simulink model "DPWMA_17_Level_Rectifier_Digital_PR"  (R2023b)
settings: Solver=VariableStepAuto  StartTime=0.0  StopTime=0.5  RelTol=1e-3
libraries: spsDiodeLib x144, spsSeriesRLCBranchLib x39, spsVoltageMeasurementLib x27, spsIGBTDiodeLib x24, simulink x12, spsACVoltageSourceLib x3, spsCurrentMeasurementLib x2, spsMeanLib x2, spsRMSLib x2, slpidlib x1, spsTHDLib x1, spspowerguiLib x1
(part 1 of 2)
settings Model: SimulationMode=accelerator  Creator=abc68  LastModifiedBy=Qu
settings DebuggingCC: UnconnectedInputMsg=warning  UnconnectedOutputMsg=warning  UnconnectedLineMsg=warning
settings ModelReferenceCC: EnableRefExpFcnMdlSchedulingChecks=on
settings RTWCC: DLArmComputeVersion=19.05

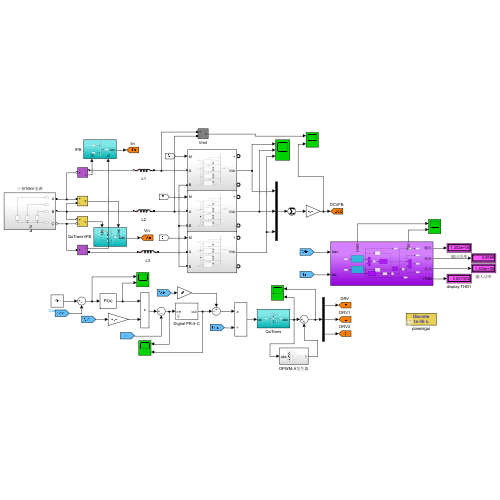
[thumbnail: Simulink's stored preview of the top-level diagram]
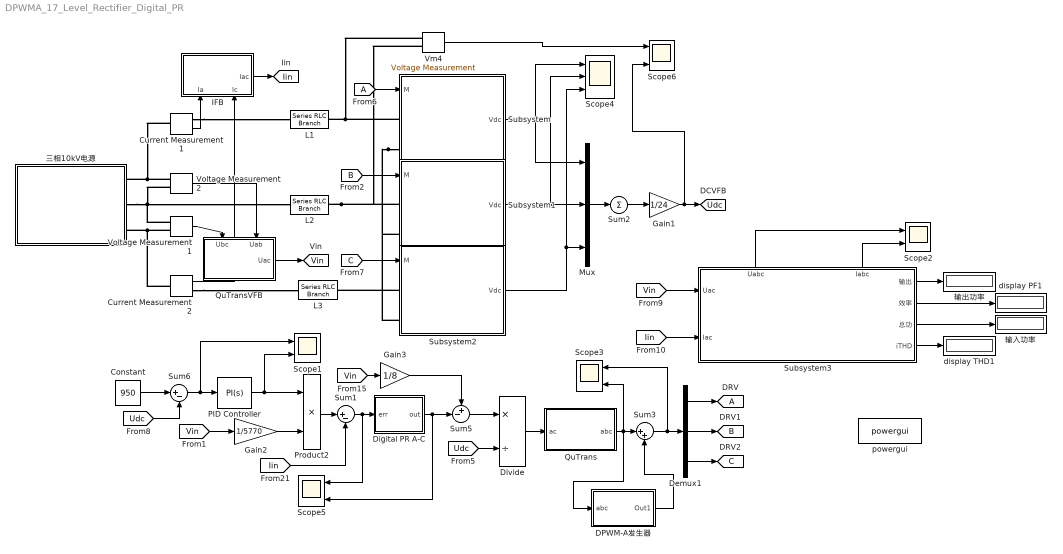
== system DPWMA_17_Level_Rectifier_Digital_PR ==
  Constant : Constant  Value=950
  Current Measurement1 : spsCurrentMeasurementLib/Current Measurement  PhasorSimulation=off  OutputType=Complex  PSBequivalent=0
  Current Measurement2 : spsCurrentMeasurementLib/Current Measurement  PhasorSimulation=off  OutputType=Complex  PSBequivalent=0
  DPWM-A发生器 : Subsystem
  DRV : Goto  TagVisibility=global
  Demux1 : Demux  Outputs=3
  Digital PR A-C : Subsystem  mask{Kp=3, Kr=30, Wc=5, Ts=1/28800, Upper=3000, Lower=-3000}
      mask DialogControl ParameterGroupVar Prompt: 参数
  Divide : Product  Inputs=*/
  From6 : From  TagVisibility=global
  Gain1 : Gain  Gain=1/24
  Gain2 : Gain  Gain=1/5770
  Gain3 : Gain  Gain=1/8
  IFB : Subsystem
      settings: PortSchema="{\"entries\":[{\"content\":{\"sides\":[{\"content\":{\"connectorIds\":[]},\"type\":\"ConnectorPlacement.EquallySpacedRectSide\",\"uuid\":\"58c40194-9a95-4e39-952e-f878bde7484e\"},{\"content\":{\"connectorIds\":[\"In1\",\"In2\"],\"side\":\"RIGHT\"},\"type\":\"ConnectorPlacement.EquallySpacedRectSide\",\"uuid\":\"f51692e8-3ff2-4d72-808d-3667196a4526\"},{\"content\":{\"connectorIds\":[],\"side\":\"TOP\"},\"type\":\"ConnectorPlacement.EquallySpacedRectSide\",\"uuid\":\"0aab136b-5da5-45c4-8998-999ebe8b7f2f\"},{\"content\":{\"connectorIds\":[\"Out1\"],\"side\":\"BOTTOM\"},\"type\":\"ConnectorPlacement.EquallySpacedRectSide\",\"uuid\":\"32f5f4a5-4ebb-496b-828d-b973bd46b44e\"}]},\"type\":\"ConnectorPlacement.EquallySpacedConnector\",\"uuid\":\"3ef81af7-d426-47fb-88e3-e33e58eebb83\"}],\"packageUris\":[\"http://schema.mathworks.com/mf0/Connector/R2020b\"],\"version\":\"1.0\"}"
  L1 : spsSeriesRLCBranchLib/Series RLC Branch  LConnTagsString=__new0  RConnTagsString=__new0  BranchType=L  Resistance=0.05  Inductance=5e-3  SetiL0=off  InitialCurrent=0  Capacitance=inf  Setx0=off  InitialVoltage=0  Measurements=None
  L2 : spsSeriesRLCBranchLib/Series RLC Branch  LConnTagsString=__new0  RConnTagsString=__new0  BranchType=L  Resistance=0.05  Inductance=5e-3  SetiL0=off  InitialCurrent=0  Capacitance=inf  Setx0=off  InitialVoltage=0  Measurements=None
  L3 : spsSeriesRLCBranchLib/Series RLC Branch  LConnTagsString=__new0  RConnTagsString=__new0  BranchType=L  Resistance=0.05  Inductance=5e-3  SetiL0=off  InitialCurrent=0  Capacitance=inf  Setx0=off  InitialVoltage=0  Measurements=None
  Mux : Mux  Inputs=3
  PID Controller : slpidlib/PID Controller  Controller=PI  Form=Parallel  TimeDomain=Continuous-time  UseExternalTs=off  SampleTime=-1  IntegratorMethod=Forward Euler  FilterMethod=Forward Euler  ControllerParametersSource=internal  P=1.5  I=120  UseKiTs=off  D=0.005  N=100  UseFilter=on  TunerSelectOption=Transfer Function Based (PID Tuner App)  InitialConditionSource=internal  InitialConditionForIntegrator=0  InitialConditionForFilter=0  DifferentiatorICPrevScaledInput=0  ExternalReset=none  TrackingMode=off  Kt=1  LimitOutput=off  SatLimitsSource=internal  UpperSaturationLimit=200  LowerSaturationLimit=0  LinearizeAsGain=on  AntiWindupMode=clamping  Kb=1  LimitIntegrator=off  UpperIntegratorSaturationLimit=inf  LowerIntegratorSaturationLimit=-inf  POutMin=[]  POutMax=[]  IOutMin=[]  IOutMax=[]  DOutMin=[]  DOutMax=[]  NOutMin=[]  NOutMax=[]  SumOutMin=[]  SumOutMax=[]  SaturationOutMin=[]  SaturationOutMax=[]  PParamMin=[]  PParamMax=[]  IParamMin=[]  IParamMax=[]  DParamMin=[]  DParamMax=[]  NParamMin=[]  NParamMax=[]  KbParamMin=[]  KbParamMax=[]  KtParamMin=[]  KtParamMax=[]  KbOutMin=[]  KbOutMax=[]  KtOutMin=[]  KtOutMax=[]  IntegratorOutMin=[]  IntegratorOutMax=[]  FilterOutMin=[]  FilterOutMax=[]  SumI1OutMin=[]  SumI1OutMax=[]  SumI2OutMin=[]  SumI2OutMax=[]  SumI3OutMin=[]  SumI3OutMax=[]  SumI4OutMin=[]  SumI4OutMax=[]  SumDOutMin=[]  SumDOutMax=[]  DifferentiatorOutMin=[]  DifferentiatorOutMax=[]  FilterDiffOutCoefMin=[]  FilterDiffOutCoefMax=[]  ReciprocalOutMin=[]  ReciprocalOutMax=[]  SumDenOutMin=[]  SumDenOutMax=[]  SumNumOutMin=[]  SumNumOutMax=[]  DivideOutMin=[]  DivideOutMax=[]  UdiffTsProdOutMin=[]  UdiffTsProdOutMax=[]  NTsProdOutMin=[]  NTsProdOutMax=[]  UintegralTsProdOutMin=[]  UintegralTsProdOutMax=[]  UngainTsProdOutMin=[]  UngainTsProdOutMax=[]  ClampingZeroOutDataTypeStr=Inherit: Inherit via back propagation  ClampingZeroOutMin=[]  ClampingZeroOutMax=[]  FilterDenConstantOutDataTypeStr=Inherit: Inherit via back propagation  FilterDenConstantOutMin=[]  FilterDenConstantOutMax=[]  PCopyOutDataTypeStr=Inherit: Inherit via back propagation  PCopyOutMin=[]  PCopyOutMax=[]  NCopyOutDataTypeStr=Inherit: Inherit via back propagation  NCopyOutMin=[]  NCopyOutMax=[]  IntegratorContinuousStateAttributes=''  IntegratorStateMustResolveToSignalObject=off  IntegratorRTWStateStorageClass=Auto  FilterContinuousStateAttributes=''  FilterStateMustResolveToSignalObject=off  FilterRTWStateStorageClass=Auto  ParallelPVariant=InternalParameters  IdealPVariant=Disabled  IVariant=InternalParameters  DVariant=Disabled  IntegratorVariant=Continuous  SatVariant=Disabled  AWVariant=Passthrough  PCopyVariant=Disabled  TRVariant=Disabled  FdbkBlocksVariant=Forward  IdealPFdbkVariant=Disabled  SatFdbkVariant=Disabled  DerivativeFilterVariant=Disabled  NVariant=Disabled  NCopyVariant=Disabled_SignalSpec  FilterICVariant=Disabled  IntegratorICVariant=InternalICs  ExternalResetVariant=Disabled  TRSumVariant=Passthrough  SumFdbkVariant=Disabled  SumVariant=Sum_PI  TsampFilterVariant=InternalTs  TsampNgainVariant=Passthrough  TsampIntegralVariant=Disabled_SignalSpec  ExternalSaturationOutDataTypeStr=Inherit: Same as second input
  Product2 : Product
  QuTrans : Subsystem
      settings: PortSchema="{\"entries\":[{\"content\":{\"sides\":[{\"content\":{\"connectorIds\":[]},\"type\":\"ConnectorPlacement.EquallySpacedRectSide\",\"uuid\":\"58c40194-9a95-4e39-952e-f878bde7484e\"},{\"content\":{\"connectorIds\":[],\"side\":\"RIGHT\"},\"type\":\"ConnectorPlacement.EquallySpacedRectSide\",\"uuid\":\"f51692e8-3ff2-4d72-808d-3667196a4526\"},{\"content\":{\"connectorIds\":[\"In1\"],\"side\":\"TOP\"},\"type\":\"ConnectorPlacement.EquallySpacedRectSide\",\"uuid\":\"0aab136b-5da5-45c4-8998-999ebe8b7f2f\"},{\"content\":{\"connectorIds\":[\"Out1\"],\"side\":\"BOTTOM\"},\"type\":\"ConnectorPlacement.EquallySpacedRectSide\",\"uuid\":\"185ce796-68e2-4136-8080-97dc86d2ba54\"}]},\"type\":\"ConnectorPlacement.EquallySpacedConnector\",\"uuid\":\"3ef81af7-d426-47fb-88e3-e33e58eebb83\"}],\"packageUris\":[\"http://schema.mathworks.com/mf0/Connector/R2020b\"],\"version\":\"1.0\"}"
  QuTransVFB : Subsystem
      settings: PortSchema="{\"entries\":[{\"content\":{\"sides\":[{\"content\":{\"connectorIds\":[\"In1\",\"In2\"]},\"type\":\"ConnectorPlacement.EquallySpacedRectSide\",\"uuid\":\"58c40194-9a95-4e39-952e-f878bde7484e\"},{\"content\":{\"connectorIds\":[],\"side\":\"RIGHT\"},\"type\":\"ConnectorPlacement.EquallySpacedRectSide\",\"uuid\":\"f51692e8-3ff2-4d72-808d-3667196a4526\"},{\"content\":{\"connectorIds\":[],\"side\":\"TOP\"},\"type\":\"ConnectorPlacement.EquallySpacedRectSide\",\"uuid\":\"0aab136b-5da5-45c4-8998-999ebe8b7f2f\"},{\"content\":{\"connectorIds\":[\"Out1\"],\"side\":\"BOTTOM\"},\"type\":\"ConnectorPlacement.EquallySpacedRectSide\",\"uuid\":\"185ce796-68e2-4136-8080-97dc86d2ba54\"}]},\"type\":\"ConnectorPlacement.EquallySpacedConnector\",\"uuid\":\"3ef81af7-d426-47fb-88e3-e33e58eebb83\"}],\"packageUris\":[\"http://schema.mathworks.com/mf0/Connector/R2020b\"],\"version\":\"1.0\"}"
  Scope{1..3,5..6} (5 alike) : Scope  NumInputPorts=2
  Scope4 : Scope  NumInputPorts=3
  Subsystem : Subsystem
      settings: PortSchema="{\"entries\":[{\"content\":{\"sides\":[{\"content\":{\"connectorIds\":[\"In1\",\"LConn1\",\"LConn2\"]},\"type\":\"ConnectorPlacement.EquallySpacedRectSide\",\"uuid\":\"5087c15a-4ffd-4c0a-98d3-826831d4ce75\"},{\"content\":{\"connectorIds\":[\"RConn1\",\"Out1\",\"RConn2\"],\"side\":\"RIGHT\"},\"type\":\"ConnectorPlacement.EquallySpacedRectSide\",\"uuid\":\"4c5a42c4-5614-4600-94e6-31252d48b405\"},{\"content\":{\"connectorIds\":[],\"side\":\"TOP\"},\"type\":\"ConnectorPlacement.EquallySpacedRectSide\",\"uuid\":\"651e2eb8-0e08-443f-8196-9bc13f283c8d\"}]},\"type\":\"ConnectorPlacement.EquallySpacedConnector\",\"uuid\":\"c413f1a7-d7be-4c94-b554-ce5b8ede92cd\"}],\"packageUris\":[\"http://schema.mathworks.com/mf0/Connector/R2020b\"],\"version\":\"1.0\"}"
  Subsystem1 : Subsystem
      settings: PortSchema="{\"entries\":[{\"content\":{\"sides\":[{\"content\":{\"connectorIds\":[\"In1\",\"LConn1\",\"LConn2\"]},\"type\":\"ConnectorPlacement.EquallySpacedRectSide\",\"uuid\":\"5087c15a-4ffd-4c0a-98d3-826831d4ce75\"},{\"content\":{\"connectorIds\":[\"RConn1\",\"Out1\",\"RConn2\"],\"side\":\"RIGHT\"},\"type\":\"ConnectorPlacement.EquallySpacedRectSide\",\"uuid\":\"4c5a42c4-5614-4600-94e6-31252d48b405\"},{\"content\":{\"connectorIds\":[],\"side\":\"TOP\"},\"type\":\"ConnectorPlacement.EquallySpacedRectSide\",\"uuid\":\"651e2eb8-0e08-443f-8196-9bc13f283c8d\"}]},\"type\":\"ConnectorPlacement.EquallySpacedConnector\",\"uuid\":\"c413f1a7-d7be-4c94-b554-ce5b8ede92cd\"}],\"packageUris\":[\"http://schema.mathworks.com/mf0/Connector/R2020b\"],\"version\":\"1.0\"}"
  Subsystem2 : Subsystem
      settings: PortSchema="{\"entries\":[{\"content\":{\"sides\":[{\"content\":{\"connectorIds\":[\"In1\",\"LConn1\",\"LConn2\"]},\"type\":\"ConnectorPlacement.EquallySpacedRectSide\",\"uuid\":\"5087c15a-4ffd-4c0a-98d3-826831d4ce75\"},{\"content\":{\"connectorIds\":[\"RConn1\",\"Out1\",\"RConn2\"],\"side\":\"RIGHT\"},\"type\":\"ConnectorPlacement.EquallySpacedRectSide\",\"uuid\":\"4c5a42c4-5614-4600-94e6-31252d48b405\"},{\"content\":{\"connectorIds\":[],\"side\":\"TOP\"},\"type\":\"ConnectorPlacement.EquallySpacedRectSide\",\"uuid\":\"651e2eb8-0e08-443f-8196-9bc13f283c8d\"}]},\"type\":\"ConnectorPlacement.EquallySpacedConnector\",\"uuid\":\"c413f1a7-d7be-4c94-b554-ce5b8ede92cd\"}],\"packageUris\":[\"http://schema.mathworks.com/mf0/Connector/R2020b\"],\"version\":\"1.0\"}"
  Subsystem3 : Subsystem
      settings: PortSchema="{\"entries\":[{\"content\":{\"sides\":[{\"content\":{\"connectorIds\":[\"In1\",\"In2\"]},\"type\":\"ConnectorPlacement.EquallySpacedRectSide\",\"uuid\":\"585310f4-b3bf-492d-9f33-7dcd19e8f218\"},{\"content\":{\"connectorIds\":[\"Out1\",\"Out2\",\"Out3\",\"Out4\"],\"side\":\"RIGHT\"},\"type\":\"ConnectorPlacement.EquallySpacedRectSide\",\"uuid\":\"5474c482-d360-4f44-8814-643502559dad\"},{\"content\":{\"connectorIds\":[\"Out5\",\"Out6\"],\"side\":\"TOP\"},\"type\":\"ConnectorPlacement.EquallySpacedRectSide\",\"uuid\":\"e6db1865-f914-4715-b807-783a3e509643\"}]},\"type\":\"ConnectorPlacement.EquallySpacedConnector\",\"uuid\":\"2bc4af52-a60f-458b-9c00-82a0e2091d31\"}],\"packageUris\":[\"http://schema.mathworks.com/mf0/Connector/R2020b\"],\"version\":\"1.0\"}"
  Sum1 : Sum  Inputs=|+-
  Sum2 : Sum  Inputs=+
  Sum3 : Sum  Inputs=|++
  Sum5 : Sum  Inputs=+-|
  Sum6 : Sum  Inputs=|+-
  Vm4 : spsVoltageMeasurementLib/Voltage Measurement  PhasorSimulation=off  OutputType=Complex  PSBequivalent=0
  Voltage Measurement1 : spsVoltageMeasurementLib/Voltage Measurement  PhasorSimulation=off  OutputType=Complex  PSBequivalent=0
  Voltage Measurement2 : spsVoltageMeasurementLib/Voltage Measurement  PhasorSimulation=off  OutputType=Complex  PSBequivalent=0
  display PF1 : Display
  display THD1 : Display
  powergui : spspowerguiLib/powergui  SimulationMode=Discrete  SampleTime=1e-6  frequency=60  Iterations=50  frequencyindice=0  Pbase=100e6  ErrMax=1e-4  UnitsV=kV  UnitsW=MW  buscounter=0  FunctionMessages=off  echomessages=off  EnableUseOfTLC=off  CurrentSourceSwitches=off  DisableSnubberDevices=off  DisableRonSwitches=off  DisableVfSwitches=off  DisplayEquations=off  AutomaticDiscreteSolvers=off  SolverType=Tustin/Backward Euler (TBE)  Interpol=off  ExternalGateDelay=off  methode=off  Ts=0  x0status=blocks  SPID=off  SwTol=0  HookPort=off  NonlinearTolerance=1e-4  nMaxIteration=100  ContinueOnMaxIteration=off  RestoreLinks=warning  ResistiveCurrentMeasurement=off  Frange=[0:2:500]  Ylog=off  Xlog=on  ShowGrid=off  save=off  variable=ZData  structure=QQQQQ  ZoomFFT=off  StartTime=0.5  cycles=15  DisplayStyle=1  fundamental=50  FreqAxis=off  MaxFrequency=1000  frequencyindicesteady=1  RmsSteady=1  display=off
  三相10kV电源 : Subsystem
      settings: PortSchema="{\"entries\":[{\"content\":{\"sides\":[{\"content\":{\"connectorIds\":[]},\"type\":\"ConnectorPlacement.EquallySpacedRectSide\",\"uuid\":\"5692784f-1b55-4d91-979b-6d4f0f069822\"},{\"content\":{\"connectorIds\":[\"RConn1\",\"RConn2\",\"RConn3\"],\"side\":\"RIGHT\"},\"type\":\"ConnectorPlacement.EquallySpacedRectSide\",\"uuid\":\"9a030936-b32a-4f05-b3f8-cc4c8aa25605\"},{\"content\":{\"connectorIds\":[],\"side\":\"TOP\"},\"type\":\"ConnectorPlacement.EquallySpacedRectSide\",\"uuid\":\"5cfc997e-60a4-43d8-bb4b-1dd6701aa9aa\"},{\"content\":{\"connectorIds\":[\"RConn4\"],\"side\":\"BOTTOM\"},\"type\":\"ConnectorPlacement.EquallySpacedRectSide\",\"uuid\":\"c52a786f-991d-42ea-bd6e-73a9c9371acb\"}]},\"type\":\"ConnectorPlacement.EquallySpacedConnector\",\"uuid\":\"853efb3d-2dc6-42ad-992e-f1defcaa0d46\"}],\"packageUris\":[\"http://schema.mathworks.com/mf0/Connector/R2020b\"],\"version\":\"1.0\"}"
  输入功率 : Display
  输出功率 : Display
  tag scope: B=global, C=global, Iin=global, Udc=global, Vin=global
  wires:
  Constant/1 -> Sum6/1
  Sum6/1 -> PID Controller/1, Scope1/1
  [Udc] -> Sum6/2
  From6/1 -> Subsystem/1(M)
  Vm4/1 -> Scope6/1
  Sum2/1 -> Gain1/1
  Gain1/1 -> Scope6/2, [Udc]
  [Vin] -> Gain2/1
  Gain2/1 -> Product2/2
  Sum1/1 -> Scope5/1, Digital PR A-C/1(err)
  Digital PR A-C/1(out) -> Scope5/2, Sum5/2
  Sum5/1 -> Divide/1
  [Iin] -> Sum1/2
  PID Controller/1 -> Scope1/2, Product2/1
  Product2/1 -> Sum1/1
  [Vin] -> Gain3/1
  Gain3/1 -> Sum5/1
  Subsystem/1(Vdc) -> Mux/1, Scope4/1
  Subsystem1/1(Vdc) -> Mux/2, Scope4/2
  Subsystem2/1(Vdc) -> Mux/3, Scope4/3
  Mux/1 -> Sum2/1
  [B] -> Subsystem1/1(M)
  [C] -> Subsystem2/1(M)
  Voltage Measurement1/1 -> QuTransVFB/1(Ubc)
  Voltage Measurement2/1 -> QuTransVFB/2(Uab)
  Current Measurement1/1 -> IFB/1(Ia)
  Current Measurement2/1 -> IFB/2(Ic)
  IFB/1(Iac) -> [Iin]
  QuTransVFB/1(Uac) -> [Vin]
  Subsystem3/2(效率) -> display PF1/1
  Subsystem3/3(总功) -> 输入功率/1
  Subsystem3/4(iTHD) -> display THD1/1
  [Vin] -> Subsystem3/1(Uac)
  [Iin] -> Subsystem3/2(Iac)
  Divide/1 -> QuTrans/1(ac)
  Subsystem3/1(输出) -> 输出功率/1
  [Udc] -> Divide/2
  Subsystem3/5(Uabc) -> Scope2/1
  Subsystem3/6(Iabc) -> Scope2/2
  Sum3/1 -> Scope3/1, Demux1/1
  QuTrans/1(abc) -> Scope3/2, DPWM-A发生器/1(abc), Sum3/1
  DPWM-A发生器/1(Out1) -> Sum3/2
  Demux1/1 -> DRV/1
  Demux1/2 -> [B]
  Demux1/3 -> [C]
  connections:
  三相10kV电源/RConn2 -- Voltage Measurement1/LConn1 -- Voltage Measurement2/LConn2 -- L2/LConn1
  Current Measurement1/RConn1 -- L1/LConn1
  Current Measurement1/LConn1 -- Voltage Measurement2/LConn1 -- 三相10kV电源/RConn1
  Current Measurement2/RConn1 -- L3/LConn1
  Current Measurement2/LConn1 -- Voltage Measurement1/LConn2 -- 三相10kV电源/RConn3
  Subsystem/LConn1 -- Vm4/LConn1 -- L1/RConn1
  Subsystem2/LConn1 -- L3/RConn1
  Subsystem/LConn2 -- Subsystem2/LConn2 -- Subsystem1/LConn2
  L2/RConn1 -- Subsystem1/LConn1 -- Vm4/LConn2

== system DPWMA_17_Level_Rectifier_Digital_PR/DPWM-A发生器 ==
  abc : Inport
  Constant1 : Constant
  Constant2 : Constant  Value=0
  Demux : Demux  Outputs=3
  Demux2 : Demux  Outputs=3
  Gain5 : Gain  Gain=-1
  MinMax : MinMax
  MinMax2 : MinMax
  Mux1 : Mux  Inputs=3
  Mux2 : Mux  Inputs=3
  Relational Operator2 : RelationalOperator  Operator=<=  OutDataTypeStr=boolean  InputSameDT=off
  Sum10 : Sum  Inputs=++|
  Sum11 : Sum  Inputs=++|
  Sum12 : Sum  Inputs=++|
  Sum4 : Sum  Inputs=|+-
  Sum8 : Sum  Inputs=|+-
  Sum9 : Sum  Inputs=|+-
  Switch{,1..6} (7 alike) : Switch  Criteria=u2 > Threshold  SaturateOnIntegerOverflow=off  InputSameDT=off
  Out1 : Outport
  wires:
  Switch1/1 -> Sum8/1
  Constant1/1 -> Switch5/3, Switch4/3, Switch3/3, Switch2/1, Switch1/1, Switch/1
  Constant2/1 -> Switch1/3, Switch/3, Switch2/3, Switch5/1, Switch4/1, Switch3/1
  Demux2/2 -> Sum11/1, Switch4/2
  Sum9/1 -> Mux1/3
  Switch2/1 -> Sum9/1
  MinMax/1 -> Switch6/1, Relational Operator2/1
  Relational Operator2/1 -> Switch6/2
  Mux1/1 -> MinMax/1
  Mux2/1 -> MinMax2/1
  Sum10/1 -> Mux2/1
  Sum11/1 -> Mux2/2
  Switch/1 -> Sum4/1
  Demux/1 -> Sum4/2, Switch/2
  Demux2/1 -> Sum10/1, Switch3/2
  Demux/3 -> Sum9/2, Switch2/2
  Sum12/1 -> Mux2/3
  Gain5/1 -> Switch6/3
  Switch4/1 -> Sum11/2
  Demux/2 -> Sum8/2, Switch1/2
  MinMax2/1 -> Gain5/1, Relational Operator2/2
  Switch5/1 -> Sum12/2
  Demux2/3 -> Switch5/2, Sum12/1
  Sum8/1 -> Mux1/2
  Sum4/1 -> Mux1/1
  Switch3/1 -> Sum10/2
  abc/1 -> Demux/1, Demux2/1
  Switch6/1 -> Out1/1

== system DPWMA_17_Level_Rectifier_Digital_PR/Digital PR A-C ==
  err : Inport
  Constant : Constant  Value=Kp
  Constant1 : Constant  Value=Kr
  Constant2 : Constant  Value=Wc
  Constant3 : Constant  Value=Ts
  Demux : Demux  Outputs=2
  Discrete PR : MATLAB Function  TreatAsAtomicUnit=on
  Mux : Mux  Inputs=2
  Saturation : Saturate  UpperLimit=Upper  LowerLimit=Lower
  out : Outport
  wires:
  Constant1/1 -> Discrete PR/4(Kr)
  Constant3/1 -> Discrete PR/6(Ts)
  Constant/1 -> Discrete PR/3(Kp)
  Constant2/1 -> Discrete PR/5(Wc)
  Demux/1 -> Discrete PR/1(err_A)
  err/1 -> Demux/1
  Demux/2 -> Discrete PR/2(err_C)
  Discrete PR/1(out_A) -> Mux/1
  Discrete PR/2(out_C) -> Mux/2
  Mux/1 -> out/1

== system DPWMA_17_Level_Rectifier_Digital_PR/IFB ==
  Ia : Inport
  Ic : Inport  Port=2
  Mux : Mux  Inputs=2
  Iac : Outport
  wires:
  Ia/1 -> Mux/1
  Ic/1 -> Mux/2
  Mux/1 -> Iac/1

== system DPWMA_17_Level_Rectifier_Digital_PR/QuTrans ==
  ac : Inport
  Demux : Demux  Outputs=2
  Mux : Mux  Inputs=3
  Sum6 : Sum  Inputs=-|-
  abc : Outport
  wires:
  ac/1 -> Demux/1
  Sum6/1 -> Mux/2
  Demux/1 -> Sum6/1, Mux/1
  Demux/2 -> Sum6/2, Mux/3
  Mux/1 -> abc/1

== system DPWMA_17_Level_Rectifier_Digital_PR/QuTransVFB ==
  Ubc : Inport
  Uab : Inport  Port=2
  Gain1 : Gain  Gain=1/3
  Gain3 : Gain  Gain=2
  Gain4 : Gain  Gain=2
  Mux : Mux  Inputs=2
  Sum2 : Sum  Inputs=--|
  Sum6 : Sum  Inputs=|++
  Uac : Outport
  wires:
  Uab/1 -> Sum2/2, Gain4/1
  Gain4/1 -> Sum6/1
  Ubc/1 -> Sum6/2, Gain3/1
  Gain3/1 -> Sum2/1
  Sum2/1 -> Mux/2
  Sum6/1 -> Mux/1
  Mux/1 -> Gain1/1
  Gain1/1 -> Uac/1

== system DPWMA_17_Level_Rectifier_Digital_PR/Subsystem ==
  M : Inport
  Mux : Mux
  子模块1 : Subsystem
      settings: PortSchema="{\"entries\":[{\"content\":{\"sides\":[{\"content\":{\"connectorIds\":[\"LConn1\",\"LConn2\"]},\"type\":\"ConnectorPlacement.EquallySpacedRectSide\",\"uuid\":\"47187a24-6853-42ac-9ad9-0df0e1360fae\"},{\"content\":{\"connectorIds\":[\"RConn1\",\"In1\",\"RConn2\"],\"side\":\"RIGHT\"},\"type\":\"ConnectorPlacement.EquallySpacedRectSide\",\"uuid\":\"b3504369-b235-4116-9b9b-167bd6b76527\"},{\"content\":{\"connectorIds\":[\"Out1\"],\"side\":\"TOP\"},\"type\":\"ConnectorPlacement.EquallySpacedRectSide\",\"uuid\":\"5cb205b4-da18-4f20-b3d4-22846a9c2236\"},{\"content\":{\"connectorIds\":[],\"side\":\"BOTTOM\"},\"type\":\"ConnectorPlacement.EquallySpacedRectSide\",\"uuid\":\"4e548a82-6bdf-470e-8572-00c7c8855d01\"}]},\"type\":\"ConnectorPlacement.EquallySpacedConnector\",\"uuid\":\"b00ba750-ea4b-4b64-a122-5cbc9e899126\"}],\"packageUris\":[\"http://schema.mathworks.com/mf0/Connector/R2020b\"],\"version\":\"1.0\"}"
  子模块2 : Subsystem
      settings: PortSchema="{\"entries\":[{\"content\":{\"sides\":[{\"content\":{\"connectorIds\":[\"LConn1\",\"LConn2\"]},\"type\":\"ConnectorPlacement.EquallySpacedRectSide\",\"uuid\":\"47187a24-6853-42ac-9ad9-0df0e1360fae\"},{\"content\":{\"connectorIds\":[\"RConn1\",\"In1\",\"RConn2\"],\"side\":\"RIGHT\"},\"type\":\"ConnectorPlacement.EquallySpacedRectSide\",\"uuid\":\"b3504369-b235-4116-9b9b-167bd6b76527\"},{\"content\":{\"connectorIds\":[\"Out1\"],\"side\":\"TOP\"},\"type\":\"ConnectorPlacement.EquallySpacedRectSide\",\"uuid\":\"5cb205b4-da18-4f20-b3d4-22846a9c2236\"},{\"content\":{\"connectorIds\":[],\"side\":\"BOTTOM\"},\"type\":\"ConnectorPlacement.EquallySpacedRectSide\",\"uuid\":\"4e548a82-6bdf-470e-8572-00c7c8855d01\"}]},\"type\":\"ConnectorPlacement.EquallySpacedConnector\",\"uuid\":\"b00ba750-ea4b-4b64-a122-5cbc9e899126\"}],\"packageUris\":[\"http://schema.mathworks.com/mf0/Connector/R2020b\"],\"version\":\"1.0\"}"
  子模块3 : Subsystem
      settings: PortSchema="{\"entries\":[{\"content\":{\"sides\":[{\"content\":{\"connectorIds\":[\"LConn1\",\"LConn2\"]},\"type\":\"ConnectorPlacement.EquallySpacedRectSide\",\"uuid\":\"47187a24-6853-42ac-9ad9-0df0e1360fae\"},{\"content\":{\"connectorIds\":[\"RConn1\",\"In1\",\"RConn2\"],\"side\":\"RIGHT\"},\"type\":\"ConnectorPlacement.EquallySpacedRectSide\",\"uuid\":\"b3504369-b235-4116-9b9b-167bd6b76527\"},{\"content\":{\"connectorIds\":[\"Out1\"],\"side\":\"TOP\"},\"type\":\"ConnectorPlacement.EquallySpacedRectSide\",\"uuid\":\"5cb205b4-da18-4f20-b3d4-22846a9c2236\"},{\"content\":{\"connectorIds\":[],\"side\":\"BOTTOM\"},\"type\":\"ConnectorPlacement.EquallySpacedRectSide\",\"uuid\":\"4e548a82-6bdf-470e-8572-00c7c8855d01\"}]},\"type\":\"ConnectorPlacement.EquallySpacedConnector\",\"uuid\":\"b00ba750-ea4b-4b64-a122-5cbc9e899126\"}],\"packageUris\":[\"http://schema.mathworks.com/mf0/Connector/R2020b\"],\"version\":\"1.0\"}"
  子模块4 : Subsystem
      settings: PortSchema="{\"entries\":[{\"content\":{\"sides\":[{\"content\":{\"connectorIds\":[\"LConn1\",\"LConn2\"]},\"type\":\"ConnectorPlacement.EquallySpacedRectSide\",\"uuid\":\"47187a24-6853-42ac-9ad9-0df0e1360fae\"},{\"content\":{\"connectorIds\":[\"RConn1\",\"In1\",\"RConn2\"],\"side\":\"RIGHT\"},\"type\":\"ConnectorPlacement.EquallySpacedRectSide\",\"uuid\":\"b3504369-b235-4116-9b9b-167bd6b76527\"},{\"content\":{\"connectorIds\":[\"Out1\"],\"side\":\"TOP\"},\"type\":\"ConnectorPlacement.EquallySpacedRectSide\",\"uuid\":\"5cb205b4-da18-4f20-b3d4-22846a9c2236\"},{\"content\":{\"connectorIds\":[],\"side\":\"BOTTOM\"},\"type\":\"ConnectorPlacement.EquallySpacedRectSide\",\"uuid\":\"4e548a82-6bdf-470e-8572-00c7c8855d01\"}]},\"type\":\"ConnectorPlacement.EquallySpacedConnector\",\"uuid\":\"b00ba750-ea4b-4b64-a122-5cbc9e899126\"}],\"packageUris\":[\"http://schema.mathworks.com/mf0/Connector/R2020b\"],\"version\":\"1.0\"}"
  A : PMIOPort  Side=Left
  B : PMIOPort  Port=2  Side=Left
  + : PMIOPort  Port=3  Side=Right
  - : PMIOPort  Port=4  Side=Right
  Vdc : Outport
  wires:
  子模块3/1(Udc) -> Mux/3
  子模块1/1(Udc) -> Mux/1
  子模块2/1(Udc) -> Mux/2
  子模块4/1(Udc) -> Mux/4
  Mux/1 -> Vdc/1
  M/1 -> 子模块2/1(M), 子模块4/1(M), 子模块3/1(M), 子模块1/1(M)
  connections:
  子模块2/RConn1 -- 子模块1/RConn2
  子模块1/RConn1 -- A/RConn1
  子模块3/RConn1 -- 子模块2/RConn2
  子模块4/RConn1 -- 子模块3/RConn2
  子模块4/RConn2 -- B/RConn1
  +/RConn1 -- 子模块1/LConn1
  -/RConn1 -- 子模块4/LConn2

== system DPWMA_17_Level_Rectifier_Digital_PR/Subsystem1 ==
  M : Inport
  Mux : Mux
  子模块1 : Subsystem
      settings: PortSchema="{\"entries\":[{\"content\":{\"sides\":[{\"content\":{\"connectorIds\":[\"LConn1\",\"LConn2\"]},\"type\":\"ConnectorPlacement.EquallySpacedRectSide\",\"uuid\":\"47187a24-6853-42ac-9ad9-0df0e1360fae\"},{\"content\":{\"connectorIds\":[\"RConn1\",\"In1\",\"RConn2\"],\"side\":\"RIGHT\"},\"type\":\"ConnectorPlacement.EquallySpacedRectSide\",\"uuid\":\"b3504369-b235-4116-9b9b-167bd6b76527\"},{\"content\":{\"connectorIds\":[\"Out1\"],\"side\":\"TOP\"},\"type\":\"ConnectorPlacement.EquallySpacedRectSide\",\"uuid\":\"5cb205b4-da18-4f20-b3d4-22846a9c2236\"},{\"content\":{\"connectorIds\":[],\"side\":\"BOTTOM\"},\"type\":\"ConnectorPlacement.EquallySpacedRectSide\",\"uuid\":\"4e548a82-6bdf-470e-8572-00c7c8855d01\"}]},\"type\":\"ConnectorPlacement.EquallySpacedConnector\",\"uuid\":\"b00ba750-ea4b-4b64-a122-5cbc9e899126\"}],\"packageUris\":[\"http://schema.mathworks.com/mf0/Connector/R2020b\"],\"version\":\"1.0\"}"
  子模块2 : Subsystem
      settings: PortSchema="{\"entries\":[{\"content\":{\"sides\":[{\"content\":{\"connectorIds\":[\"LConn1\",\"LConn2\"]},\"type\":\"ConnectorPlacement.EquallySpacedRectSide\",\"uuid\":\"47187a24-6853-42ac-9ad9-0df0e1360fae\"},{\"content\":{\"connectorIds\":[\"RConn1\",\"In1\",\"RConn2\"],\"side\":\"RIGHT\"},\"type\":\"ConnectorPlacement.EquallySpacedRectSide\",\"uuid\":\"b3504369-b235-4116-9b9b-167bd6b76527\"},{\"content\":{\"connectorIds\":[\"Out1\"],\"side\":\"TOP\"},\"type\":\"ConnectorPlacement.EquallySpacedRectSide\",\"uuid\":\"5cb205b4-da18-4f20-b3d4-22846a9c2236\"},{\"content\":{\"connectorIds\":[],\"side\":\"BOTTOM\"},\"type\":\"ConnectorPlacement.EquallySpacedRectSide\",\"uuid\":\"4e548a82-6bdf-470e-8572-00c7c8855d01\"}]},\"type\":\"ConnectorPlacement.EquallySpacedConnector\",\"uuid\":\"b00ba750-ea4b-4b64-a122-5cbc9e899126\"}],\"packageUris\":[\"http://schema.mathworks.com/mf0/Connector/R2020b\"],\"version\":\"1.0\"}"
  子模块3 : Subsystem
      settings: PortSchema="{\"entries\":[{\"content\":{\"sides\":[{\"content\":{\"connectorIds\":[\"LConn1\",\"LConn2\"]},\"type\":\"ConnectorPlacement.EquallySpacedRectSide\",\"uuid\":\"47187a24-6853-42ac-9ad9-0df0e1360fae\"},{\"content\":{\"connectorIds\":[\"RConn1\",\"In1\",\"RConn2\"],\"side\":\"RIGHT\"},\"type\":\"ConnectorPlacement.EquallySpacedRectSide\",\"uuid\":\"b3504369-b235-4116-9b9b-167bd6b76527\"},{\"content\":{\"connectorIds\":[\"Out1\"],\"side\":\"TOP\"},\"type\":\"ConnectorPlacement.EquallySpacedRectSide\",\"uuid\":\"5cb205b4-da18-4f20-b3d4-22846a9c2236\"},{\"content\":{\"connectorIds\":[],\"side\":\"BOTTOM\"},\"type\":\"ConnectorPlacement.EquallySpacedRectSide\",\"uuid\":\"4e548a82-6bdf-470e-8572-00c7c8855d01\"}]},\"type\":\"ConnectorPlacement.EquallySpacedConnector\",\"uuid\":\"b00ba750-ea4b-4b64-a122-5cbc9e899126\"}],\"packageUris\":[\"http://schema.mathworks.com/mf0/Connector/R2020b\"],\"version\":\"1.0\"}"
  子模块4 : Subsystem
      settings: PortSchema="{\"entries\":[{\"content\":{\"sides\":[{\"content\":{\"connectorIds\":[\"LConn1\",\"LConn2\"]},\"type\":\"ConnectorPlacement.EquallySpacedRectSide\",\"uuid\":\"47187a24-6853-42ac-9ad9-0df0e1360fae\"},{\"content\":{\"connectorIds\":[\"RConn1\",\"In1\",\"RConn2\"],\"side\":\"RIGHT\"},\"type\":\"ConnectorPlacement.EquallySpacedRectSide\",\"uuid\":\"b3504369-b235-4116-9b9b-167bd6b76527\"},{\"content\":{\"connectorIds\":[\"Out1\"],\"side\":\"TOP\"},\"type\":\"ConnectorPlacement.EquallySpacedRectSide\",\"uuid\":\"5cb205b4-da18-4f20-b3d4-22846a9c2236\"},{\"content\":{\"connectorIds\":[],\"side\":\"BOTTOM\"},\"type\":\"ConnectorPlacement.EquallySpacedRectSide\",\"uuid\":\"4e548a82-6bdf-470e-8572-00c7c8855d01\"}]},\"type\":\"ConnectorPlacement.EquallySpacedConnector\",\"uuid\":\"b00ba750-ea4b-4b64-a122-5cbc9e899126\"}],\"packageUris\":[\"http://schema.mathworks.com/mf0/Connector/R2020b\"],\"version\":\"1.0\"}"
  A : PMIOPort  Side=Left
  B : PMIOPort  Port=2  Side=Left
  + : PMIOPort  Port=3  Side=Right
  - : PMIOPort  Port=4  Side=Right
  Vdc : Outport
  wires:
  M/1 -> 子模块1/1(M), 子模块3/1(M), 子模块4/1(M), 子模块2/1(M)
  Mux/1 -> Vdc/1
  子模块4/1(Udc) -> Mux/4
  子模块2/1(Udc) -> Mux/2
  子模块1/1(Udc) -> Mux/1
  子模块3/1(Udc) -> Mux/3
  connections:
  -/RConn1 -- 子模块4/LConn2
  +/RConn1 -- 子模块1/LConn1
  子模块4/RConn2 -- B/RConn1
  子模块4/RConn1 -- 子模块3/RConn2
  子模块3/RConn1 -- 子模块2/RConn2
  子模块1/RConn1 -- A/RConn1
  子模块2/RConn1 -- 子模块1/RConn2

== system DPWMA_17_Level_Rectifier_Digital_PR/Subsystem2 ==
  M : Inport
  Mux : Mux
  子模块1 : Subsystem
      settings: PortSchema="{\"entries\":[{\"content\":{\"sides\":[{\"content\":{\"connectorIds\":[\"LConn1\",\"LConn2\"]},\"type\":\"ConnectorPlacement.EquallySpacedRectSide\",\"uuid\":\"47187a24-6853-42ac-9ad9-0df0e1360fae\"},{\"content\":{\"connectorIds\":[\"RConn1\",\"In1\",\"RConn2\"],\"side\":\"RIGHT\"},\"type\":\"ConnectorPlacement.EquallySpacedRectSide\",\"uuid\":\"b3504369-b235-4116-9b9b-167bd6b76527\"},{\"content\":{\"connectorIds\":[\"Out1\"],\"side\":\"TOP\"},\"type\":\"ConnectorPlacement.EquallySpacedRectSide\",\"uuid\":\"5cb205b4-da18-4f20-b3d4-22846a9c2236\"},{\"content\":{\"connectorIds\":[],\"side\":\"BOTTOM\"},\"type\":\"ConnectorPlacement.EquallySpacedRectSide\",\"uuid\":\"4e548a82-6bdf-470e-8572-00c7c8855d01\"}]},\"type\":\"ConnectorPlacement.EquallySpacedConnector\",\"uuid\":\"b00ba750-ea4b-4b64-a122-5cbc9e899126\"}],\"packageUris\":[\"http://schema.mathworks.com/mf0/Connector/R2020b\"],\"version\":\"1.0\"}"
  子模块2 : Subsystem
      settings: PortSchema="{\"entries\":[{\"content\":{\"sides\":[{\"content\":{\"connectorIds\":[\"LConn1\",\"LConn2\"]},\"type\":\"ConnectorPlacement.EquallySpacedRectSide\",\"uuid\":\"47187a24-6853-42ac-9ad9-0df0e1360fae\"},{\"content\":{\"connectorIds\":[\"RConn1\",\"In1\",\"RConn2\"],\"side\":\"RIGHT\"},\"type\":\"ConnectorPlacement.EquallySpacedRectSide\",\"uuid\":\"b3504369-b235-4116-9b9b-167bd6b76527\"},{\"content\":{\"connectorIds\":[\"Out1\"],\"side\":\"TOP\"},\"type\":\"ConnectorPlacement.EquallySpacedRectSide\",\"uuid\":\"5cb205b4-da18-4f20-b3d4-22846a9c2236\"},{\"content\":{\"connectorIds\":[],\"side\":\"BOTTOM\"},\"type\":\"ConnectorPlacement.EquallySpacedRectSide\",\"uuid\":\"4e548a82-6bdf-470e-8572-00c7c8855d01\"}]},\"type\":\"ConnectorPlacement.EquallySpacedConnector\",\"uuid\":\"b00ba750-ea4b-4b64-a122-5cbc9e899126\"}],\"packageUris\":[\"http://schema.mathworks.com/mf0/Connector/R2020b\"],\"version\":\"1.0\"}"
  子模块3 : Subsystem
      settings: PortSchema="{\"entries\":[{\"content\":{\"sides\":[{\"content\":{\"connectorIds\":[\"LConn1\",\"LConn2\"]},\"type\":\"ConnectorPlacement.EquallySpacedRectSide\",\"uuid\":\"47187a24-6853-42ac-9ad9-0df0e1360fae\"},{\"content\":{\"connectorIds\":[\"RConn1\",\"In1\",\"RConn2\"],\"side\":\"RIGHT\"},\"type\":\"ConnectorPlacement.EquallySpacedRectSide\",\"uuid\":\"b3504369-b235-4116-9b9b-167bd6b76527\"},{\"content\":{\"connectorIds\":[\"Out1\"],\"side\":\"TOP\"},\"type\":\"ConnectorPlacement.EquallySpacedRectSide\",\"uuid\":\"5cb205b4-da18-4f20-b3d4-22846a9c2236\"},{\"content\":{\"connectorIds\":[],\"side\":\"BOTTOM\"},\"type\":\"ConnectorPlacement.EquallySpacedRectSide\",\"uuid\":\"4e548a82-6bdf-470e-8572-00c7c8855d01\"}]},\"type\":\"ConnectorPlacement.EquallySpacedConnector\",\"uuid\":\"b00ba750-ea4b-4b64-a122-5cbc9e899126\"}],\"packageUris\":[\"http://schema.mathworks.com/mf0/Connector/R2020b\"],\"version\":\"1.0\"}"
  子模块4 : Subsystem
      settings: PortSchema="{\"entries\":[{\"content\":{\"sides\":[{\"content\":{\"connectorIds\":[\"LConn1\",\"LConn2\"]},\"type\":\"ConnectorPlacement.EquallySpacedRectSide\",\"uuid\":\"47187a24-6853-42ac-9ad9-0df0e1360fae\"},{\"content\":{\"connectorIds\":[\"RConn1\",\"In1\",\"RConn2\"],\"side\":\"RIGHT\"},\"type\":\"ConnectorPlacement.EquallySpacedRectSide\",\"uuid\":\"b3504369-b235-4116-9b9b-167bd6b76527\"},{\"content\":{\"connectorIds\":[\"Out1\"],\"side\":\"TOP\"},\"type\":\"ConnectorPlacement.EquallySpacedRectSide\",\"uuid\":\"5cb205b4-da18-4f20-b3d4-22846a9c2236\"},{\"content\":{\"connectorIds\":[],\"side\":\"BOTTOM\"},\"type\":\"ConnectorPlacement.EquallySpacedRectSide\",\"uuid\":\"4e548a82-6bdf-470e-8572-00c7c8855d01\"}]},\"type\":\"ConnectorPlacement.EquallySpacedConnector\",\"uuid\":\"b00ba750-ea4b-4b64-a122-5cbc9e899126\"}],\"packageUris\":[\"http://schema.mathworks.com/mf0/Connector/R2020b\"],\"version\":\"1.0\"}"
  A : PMIOPort  Side=Left
  B : PMIOPort  Port=2  Side=Left
  + : PMIOPort  Port=3  Side=Right
  - : PMIOPort  Port=4  Side=Right
  Vdc : Outport
  wires:
  子模块3/1(Udc) -> Mux/3
  子模块1/1(Udc) -> Mux/1
  子模块2/1(Udc) -> Mux/2
  子模块4/1(Udc) -> Mux/4
  Mux/1 -> Vdc/1
  M/1 -> 子模块2/1(M), 子模块4/1(M), 子模块3/1(M), 子模块1/1(M)
  connections:
  子模块2/RConn1 -- 子模块1/RConn2
  子模块1/RConn1 -- A/RConn1
  子模块3/RConn1 -- 子模块2/RConn2
  子模块4/RConn1 -- 子模块3/RConn2
  子模块4/RConn2 -- B/RConn1
  +/RConn1 -- 子模块1/LConn1
  -/RConn1 -- 子模块4/LConn2

== system DPWMA_17_Level_Rectifier_Digital_PR/Subsystem3 ==
  Uac : Inport
  Iac : Inport  Port=2
  Divide2 : Product  Inputs=*/
  Gain6 : Gain  Gain=1/3
  Mean : spsMeanLib/Mean  Freq=100  Vinit=0  Ts=0
  Mean1 : spsMeanLib/Mean  Freq=20000  Vinit=0  Ts=0
  Product2 : Product
  Product4 : Product
  QuTrans : Subsystem
      settings: PortSchema="{\"entries\":[{\"content\":{\"sides\":[{\"content\":{\"connectorIds\":[]},\"type\":\"ConnectorPlacement.EquallySpacedRectSide\",\"uuid\":\"58c40194-9a95-4e39-952e-f878bde7484e\"},{\"content\":{\"connectorIds\":[],\"side\":\"RIGHT\"},\"type\":\"ConnectorPlacement.EquallySpacedRectSide\",\"uuid\":\"f51692e8-3ff2-4d72-808d-3667196a4526\"},{\"content\":{\"connectorIds\":[\"In1\"],\"side\":\"TOP\"},\"type\":\"ConnectorPlacement.EquallySpacedRectSide\",\"uuid\":\"0aab136b-5da5-45c4-8998-999ebe8b7f2f\"},{\"content\":{\"connectorIds\":[\"Out1\"],\"side\":\"BOTTOM\"},\"type\":\"ConnectorPlacement.EquallySpacedRectSide\",\"uuid\":\"185ce796-68e2-4136-8080-97dc86d2ba54\"}]},\"type\":\"ConnectorPlacement.EquallySpacedConnector\",\"uuid\":\"3ef81af7-d426-47fb-88e3-e33e58eebb83\"}],\"packageUris\":[\"http://schema.mathworks.com/mf0/Connector/R2020b\"],\"version\":\"1.0\"}"
  QuTrans1 : Subsystem
      settings: PortSchema="{\"entries\":[{\"content\":{\"sides\":[{\"content\":{\"connectorIds\":[]},\"type\":\"ConnectorPlacement.EquallySpacedRectSide\",\"uuid\":\"58c40194-9a95-4e39-952e-f878bde7484e\"},{\"content\":{\"connectorIds\":[],\"side\":\"RIGHT\"},\"type\":\"ConnectorPlacement.EquallySpacedRectSide\",\"uuid\":\"f51692e8-3ff2-4d72-808d-3667196a4526\"},{\"content\":{\"connectorIds\":[\"In1\"],\"side\":\"TOP\"},\"type\":\"ConnectorPlacement.EquallySpacedRectSide\",\"uuid\":\"0aab136b-5da5-45c4-8998-999ebe8b7f2f\"},{\"content\":{\"connectorIds\":[\"Out1\"],\"side\":\"BOTTOM\"},\"type\":\"ConnectorPlacement.EquallySpacedRectSide\",\"uuid\":\"185ce796-68e2-4136-8080-97dc86d2ba54\"}]},\"type\":\"ConnectorPlacement.EquallySpacedConnector\",\"uuid\":\"3ef81af7-d426-47fb-88e3-e33e58eebb83\"}],\"packageUris\":[\"http://schema.mathworks.com/mf0/Connector/R2020b\"],\"version\":\"1.0\"}"
  RMS2 : spsRMSLib/RMS  TrueRMS=on  Freq=50  RMSInit=0  Ts=0
  RMS3 : spsRMSLib/RMS  TrueRMS=on  Freq=50  RMSInit=0  Ts=0
  Sum1 : Sum  Inputs=+
  Sum6 : Sum  Inputs=+
  Sum7 : Sum  Inputs=+
  THD : spsTHDLib/THD  Freq=50  Ts=0
  输出 : Outport
  效率 : Outport  Port=2
  总功 : Outport  Port=3
  iTHD : Outport  Port=4
  Uabc : Outport  Port=5
  Iabc : Outport  Port=6
  wires:
  RMS3/1 -> Product4/1
  Product4/1 -> Sum7/1
  Sum6/1 -> Mean/1
  Product2/1 -> Sum6/1
  Divide2/1 -> 效率/1
  RMS2/1 -> Product4/2
  Sum1/1 -> Gain6/1
  Gain6/1 -> iTHD/1
  Sum7/1 -> 总功/1, Divide2/2
  Mean/1 -> 输出/1, Divide2/1
  THD/1 -> Sum1/1
  Mean1/1 -> THD/1
  Uac/1 -> QuTrans/1(ac)
  Iac/1 -> QuTrans1/1(ac)
  QuTrans1/1(abc) -> Product2/2, Iabc/1, Mean1/1, RMS2/1
  QuTrans/1(abc) -> Uabc/1, RMS3/1, Product2/1

== system DPWMA_17_Level_Rectifier_Digital_PR/三相10kV电源 ==
  5.7KV2 : spsACVoltageSourceLib/AC Voltage Source  Amplitude=5770*1.414  Phase=120  Frequency=50  SampleTime=0  Measurements=None  BusType=swing  Pref=10e3  Qref=0  Qmin=-inf  Qmax=+inf
  5.7kV : spsACVoltageSourceLib/AC Voltage Source  Amplitude=5770*1.414  Phase=0  Frequency=50  SampleTime=0  Measurements=None  BusType=swing  Pref=10e3  Qref=0  Qmin=-inf  Qmax=+inf
  5.7kV1 : spsACVoltageSourceLib/AC Voltage Source  Amplitude=5770*1.414  Phase=240  Frequency=50  SampleTime=0  Measurements=None  BusType=swing  Pref=10e3  Qref=0  Qmin=-inf  Qmax=+inf
  A : PMIOPort  Side=Right
  B : PMIOPort  Port=2  Side=Right
  C : PMIOPort  Port=3  Side=Right
  N : PMIOPort  Port=4  Side=Right
  connections:
  5.7kV/LConn1 -- N/RConn1 -- 5.7KV2/LConn1 -- 5.7kV1/LConn1
  A/RConn1 -- 5.7kV/RConn1
  B/RConn1 -- 5.7kV1/RConn1
  C/RConn1 -- 5.7KV2/RConn1

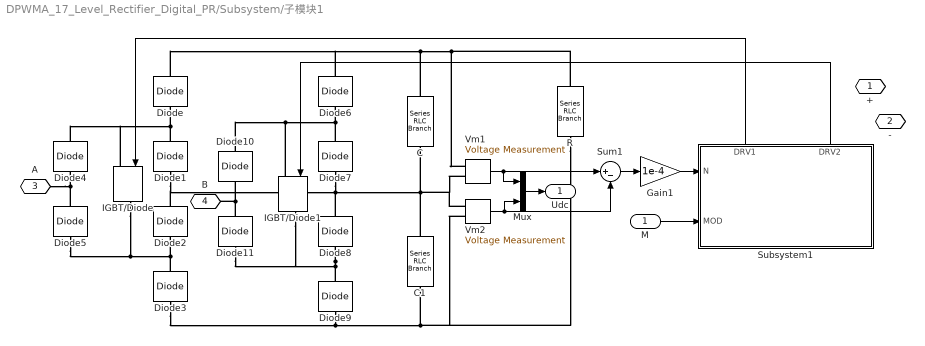
== system DPWMA_17_Level_Rectifier_Digital_PR/Subsystem/子模块1 ==
  M : Inport
  C : spsSeriesRLCBranchLib/Series RLC Branch  LConnTagsString=__new0  RConnTagsString=__new0  BranchType=C  Resistance=0  Inductance=0  SetiL0=off  InitialCurrent=0  Capacitance=4e-3  Setx0=on  InitialVoltage=860  Measurements=None
  C1 : spsSeriesRLCBranchLib/Series RLC Branch  LConnTagsString=__new0  RConnTagsString=__new0  BranchType=C  Resistance=0  Inductance=0  SetiL0=off  InitialCurrent=0  Capacitance=4e-3  Setx0=on  InitialVoltage=860  Measurements=None
  Diode{,1..3,6..9} (8 alike) : spsDiodeLib/Diode  Ron=0.001  Lon=0  Vf=1.8  IC=0  UseSnubber=0  Rs=5e6  Cs=2e-9  Measurements=off
  Diode{4..5,10..11} (4 alike) : spsDiodeLib/Diode  Ron=0.001  Lon=0  Vf=1  IC=0  UseSnubber=0  Rs=0.05  Cs=1e-8  Measurements=off
  Gain1 : Gain  Gain=1e-4
  IGBT/Diode : spsIGBTDiodeLib/IGBT//Diode  Ron=1e-3  Rs=1e5  Cs=inf  Measurements=off
  IGBT/Diode1 : spsIGBTDiodeLib/IGBT//Diode  Ron=1e-3  Rs=1e5  Cs=inf  Measurements=off
  Mux : Mux  Inputs=2
  R : spsSeriesRLCBranchLib/Series RLC Branch  LConnTagsString=__new0  RConnTagsString=__new0  BranchType=R  Resistance=30  Inductance=0  SetiL0=off  InitialCurrent=0  Capacitance=2e-3  Setx0=on  InitialVoltage=311  Measurements=None
  Subsystem1 : Subsystem
      settings: PortSchema="{\"entries\":[{\"content\":{\"sides\":[{\"content\":{\"connectorIds\":[\"In1\",\"In2\"]},\"type\":\"ConnectorPlacement.EquallySpacedRectSide\",\"uuid\":\"86aef1ad-fbca-44c0-97c4-c9d179baa788\"},{\"content\":{\"side\":\"RIGHT\"},\"type\":\"ConnectorPlacement.EquallySpacedRectSide\",\"uuid\":\"7b15a0f8-39b1-4cc5-afe7-a687626936eb\"},{\"content\":{\"connectorIds\":[\"Out1\",\"Out2\"],\"side\":\"TOP\"},\"type\":\"ConnectorPlacement.EquallySpacedRectSide\",\"uuid\":\"a58ec6d0-3129-4061-af12-e971b5e0e948\"}]},\"type\":\"ConnectorPlacement.EquallySpacedConnector\",\"uuid\":\"d3f7daee-0424-497d-bc41-11931290c6fe\"}],\"packageUris\":[\"http://schema.mathworks.com/mf0/Connector/R2020b\"],\"version\":\"1.0\"}"
  Sum1 : Sum  Inputs=|+-
  Vm1 : spsVoltageMeasurementLib/Voltage Measurement  PhasorSimulation=off  OutputType=Complex  PSBequivalent=0
  Vm2 : spsVoltageMeasurementLib/Voltage Measurement  PhasorSimulation=off  OutputType=Complex  PSBequivalent=0
  + : PMIOPort  Side=Left
  - : PMIOPort  Port=2  Side=Left
  A : PMIOPort  Port=3  Side=Right
  B : PMIOPort  Port=4  Side=Right
  Udc : Outport
  wires:
  Vm1/1 -> Mux/1, Sum1/1
  Vm2/1 -> Mux/2, Sum1/2
  Sum1/1 -> Gain1/1
  Gain1/1 -> Subsystem1/1(N)
  Mux/1 -> Udc/1
  M/1 -> Subsystem1/2(MOD)
  Subsystem1/1(DRV1) -> IGBT/Diode/1
  Subsystem1/2(DRV2) -> IGBT/Diode1/1
  connections:
  Vm1/LConn1 -- Diode6/RConn1 -- Diode/RConn1 -- C/LConn1 -- R/LConn1
  C1/LConn1 -- Diode7/LConn1 -- Diode8/RConn1 -- Diode1/LConn1 -- Diode2/RConn1 -- Vm1/LConn2 -- Vm2/LConn1 -- C/RConn1
  Diode1/RConn1 -- Diode4/RConn1 -- IGBT/Diode/LConn1 -- Diode/LConn1
  IGBT/Diode/RConn1 -- Diode5/LConn1 -- Diode2/LConn1 -- Diode3/RConn1
  Diode3/LConn1 -- Diode9/LConn1 -- R/RConn1 -- Vm2/LConn2 -- C1/RConn1
  Diode5/RConn1 -- A/RConn1 -- Diode4/LConn1
  Diode10/RConn1 -- IGBT/Diode1/LConn1 -- Diode7/RConn1 -- Diode6/LConn1
  Diode8/LConn1 -- Diode9/RConn1 -- Diode11/LConn1 -- IGBT/Diode1/RConn1
  Diode11/RConn1 -- Diode10/LConn1 -- B/RConn1

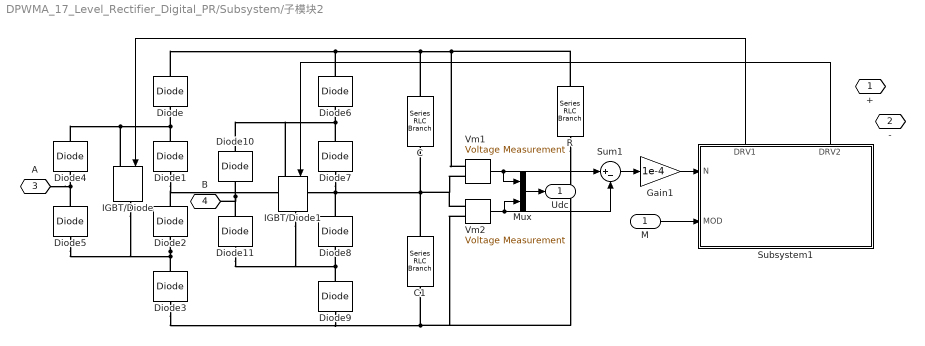
== system DPWMA_17_Level_Rectifier_Digital_PR/Subsystem/子模块2 ==
  M : Inport
  C : spsSeriesRLCBranchLib/Series RLC Branch  LConnTagsString=__new0  RConnTagsString=__new0  BranchType=C  Resistance=0  Inductance=0  SetiL0=off  InitialCurrent=0  Capacitance=4e-3  Setx0=on  InitialVoltage=850  Measurements=None
  C1 : spsSeriesRLCBranchLib/Series RLC Branch  LConnTagsString=__new0  RConnTagsString=__new0  BranchType=C  Resistance=0  Inductance=0  SetiL0=off  InitialCurrent=0  Capacitance=4e-3  Setx0=on  InitialVoltage=850  Measurements=None
  Diode{,1..3,6..9} (8 alike) : spsDiodeLib/Diode  Ron=0.001  Lon=0  Vf=1.8  IC=0  UseSnubber=0  Rs=5e6  Cs=2e-9  Measurements=off
  Diode{4..5,10..11} (4 alike) : spsDiodeLib/Diode  Ron=0.001  Lon=0  Vf=1  IC=0  UseSnubber=0  Rs=0.05  Cs=1e-8  Measurements=off
  Gain1 : Gain  Gain=1e-4
  IGBT/Diode : spsIGBTDiodeLib/IGBT//Diode  Ron=1e-3  Rs=1e5  Cs=inf  Measurements=off
  IGBT/Diode1 : spsIGBTDiodeLib/IGBT//Diode  Ron=1e-3  Rs=1e5  Cs=inf  Measurements=off
  Mux : Mux  Inputs=2
  R : spsSeriesRLCBranchLib/Series RLC Branch  LConnTagsString=__new0  RConnTagsString=__new0  BranchType=R  Resistance=30  Inductance=0  SetiL0=off  InitialCurrent=0  Capacitance=2e-3  Setx0=on  InitialVoltage=311  Measurements=None
  Subsystem1 : Subsystem
      settings: PortSchema="{\"entries\":[{\"content\":{\"sides\":[{\"content\":{\"connectorIds\":[\"In1\",\"In2\"]},\"type\":\"ConnectorPlacement.EquallySpacedRectSide\",\"uuid\":\"86aef1ad-fbca-44c0-97c4-c9d179baa788\"},{\"content\":{\"side\":\"RIGHT\"},\"type\":\"ConnectorPlacement.EquallySpacedRectSide\",\"uuid\":\"7b15a0f8-39b1-4cc5-afe7-a687626936eb\"},{\"content\":{\"connectorIds\":[\"Out1\",\"Out2\"],\"side\":\"TOP\"},\"type\":\"ConnectorPlacement.EquallySpacedRectSide\",\"uuid\":\"a58ec6d0-3129-4061-af12-e971b5e0e948\"}]},\"type\":\"ConnectorPlacement.EquallySpacedConnector\",\"uuid\":\"d3f7daee-0424-497d-bc41-11931290c6fe\"}],\"packageUris\":[\"http://schema.mathworks.com/mf0/Connector/R2020b\"],\"version\":\"1.0\"}"
  Sum1 : Sum  Inputs=|+-
  Vm1 : spsVoltageMeasurementLib/Voltage Measurement  PhasorSimulation=off  OutputType=Complex  PSBequivalent=0
  Vm2 : spsVoltageMeasurementLib/Voltage Measurement  PhasorSimulation=off  OutputType=Complex  PSBequivalent=0
  + : PMIOPort  Side=Left
  - : PMIOPort  Port=2  Side=Left
  A : PMIOPort  Port=3  Side=Right
  B : PMIOPort  Port=4  Side=Right
  Udc : Outport
  wires:
  Subsystem1/2(DRV2) -> IGBT/Diode1/1
  Subsystem1/1(DRV1) -> IGBT/Diode/1
  M/1 -> Subsystem1/2(MOD)
  Mux/1 -> Udc/1
  Gain1/1 -> Subsystem1/1(N)
  Sum1/1 -> Gain1/1
  Vm2/1 -> Sum1/2, Mux/2
  Vm1/1 -> Sum1/1, Mux/1
  connections:
  Diode10/LConn1 -- B/RConn1 -- Diode11/RConn1
  Diode9/RConn1 -- Diode8/LConn1 -- IGBT/Diode1/RConn1 -- Diode11/LConn1
  Diode7/RConn1 -- Diode6/LConn1 -- Diode10/RConn1 -- IGBT/Diode1/LConn1
  A/RConn1 -- Diode5/RConn1 -- Diode4/LConn1
  Vm2/LConn2 -- R/RConn1 -- Diode3/LConn1 -- Diode9/LConn1 -- C1/RConn1
  Diode2/LConn1 -- Diode3/RConn1 -- Diode5/LConn1 -- IGBT/Diode/RConn1
  Diode4/RConn1 -- IGBT/Diode/LConn1 -- Diode1/RConn1 -- Diode/LConn1
  Diode7/LConn1 -- Diode2/RConn1 -- Diode1/LConn1 -- C/RConn1 -- C1/LConn1 -- Vm2/LConn1 -- Vm1/LConn2 -- Diode8/RConn1
  Diode6/RConn1 -- Diode/RConn1 -- C/LConn1 -- R/LConn1 -- Vm1/LConn1

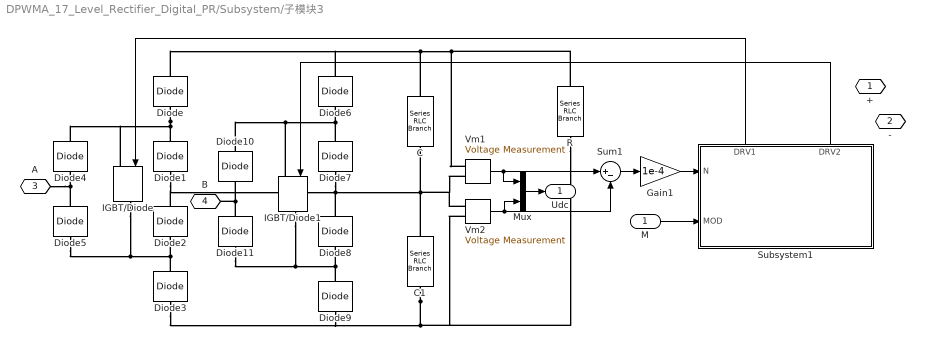
== system DPWMA_17_Level_Rectifier_Digital_PR/Subsystem/子模块3 ==
  M : Inport
  C : spsSeriesRLCBranchLib/Series RLC Branch  LConnTagsString=__new0  RConnTagsString=__new0  BranchType=C  Resistance=0  Inductance=0  SetiL0=off  InitialCurrent=0  Capacitance=4e-3  Setx0=on  InitialVoltage=850  Measurements=None
  C1 : spsSeriesRLCBranchLib/Series RLC Branch  LConnTagsString=__new0  RConnTagsString=__new0  BranchType=C  Resistance=0  Inductance=0  SetiL0=off  InitialCurrent=0  Capacitance=4e-3  Setx0=on  InitialVoltage=850  Measurements=None
  Diode{,1..3,6..9} (8 alike) : spsDiodeLib/Diode  Ron=0.001  Lon=0  Vf=1.8  IC=0  UseSnubber=0  Rs=5e6  Cs=2e-9  Measurements=off
  Diode{4..5,10..11} (4 alike) : spsDiodeLib/Diode  Ron=0.001  Lon=0  Vf=1  IC=0  UseSnubber=0  Rs=0.05  Cs=1e-8  Measurements=off
  Gain1 : Gain  Gain=1e-4
  IGBT/Diode : spsIGBTDiodeLib/IGBT//Diode  Ron=1e-3  Rs=1e5  Cs=inf  Measurements=off
  IGBT/Diode1 : spsIGBTDiodeLib/IGBT//Diode  Ron=1e-3  Rs=1e5  Cs=inf  Measurements=off
  Mux : Mux  Inputs=2
  R : spsSeriesRLCBranchLib/Series RLC Branch  LConnTagsString=__new0  RConnTagsString=__new0  BranchType=R  Resistance=30  Inductance=0  SetiL0=off  InitialCurrent=0  Capacitance=2e-3  Setx0=on  InitialVoltage=311  Measurements=None
  Subsystem1 : Subsystem
      settings: PortSchema="{\"entries\":[{\"content\":{\"sides\":[{\"content\":{\"connectorIds\":[\"In1\",\"In2\"]},\"type\":\"ConnectorPlacement.EquallySpacedRectSide\",\"uuid\":\"86aef1ad-fbca-44c0-97c4-c9d179baa788\"},{\"content\":{\"side\":\"RIGHT\"},\"type\":\"ConnectorPlacement.EquallySpacedRectSide\",\"uuid\":\"7b15a0f8-39b1-4cc5-afe7-a687626936eb\"},{\"content\":{\"connectorIds\":[\"Out1\",\"Out2\"],\"side\":\"TOP\"},\"type\":\"ConnectorPlacement.EquallySpacedRectSide\",\"uuid\":\"a58ec6d0-3129-4061-af12-e971b5e0e948\"}]},\"type\":\"ConnectorPlacement.EquallySpacedConnector\",\"uuid\":\"d3f7daee-0424-497d-bc41-11931290c6fe\"}],\"packageUris\":[\"http://schema.mathworks.com/mf0/Connector/R2020b\"],\"version\":\"1.0\"}"
  Sum1 : Sum  Inputs=|+-
  Vm1 : spsVoltageMeasurementLib/Voltage Measurement  PhasorSimulation=off  OutputType=Complex  PSBequivalent=0
  Vm2 : spsVoltageMeasurementLib/Voltage Measurement  PhasorSimulation=off  OutputType=Complex  PSBequivalent=0
  + : PMIOPort  Side=Left
  - : PMIOPort  Port=2  Side=Left
  A : PMIOPort  Port=3  Side=Right
  B : PMIOPort  Port=4  Side=Right
  Udc : Outport
  wires:
  Vm1/1 -> Mux/1, Sum1/1
  Vm2/1 -> Mux/2, Sum1/2
  Sum1/1 -> Gain1/1
  Gain1/1 -> Subsystem1/1(N)
  Mux/1 -> Udc/1
  M/1 -> Subsystem1/2(MOD)
  Subsystem1/1(DRV1) -> IGBT/Diode/1
  Subsystem1/2(DRV2) -> IGBT/Diode1/1
  connections:
  Vm1/LConn1 -- R/LConn1 -- C/LConn1 -- Diode/RConn1 -- Diode6/RConn1
  Diode8/RConn1 -- Vm1/LConn2 -- Vm2/LConn1 -- C1/LConn1 -- C/RConn1 -- Diode1/LConn1 -- Diode2/RConn1 -- Diode7/LConn1
  Diode/LConn1 -- Diode1/RConn1 -- IGBT/Diode/LConn1 -- Diode4/RConn1
  IGBT/Diode/RConn1 -- Diode5/LConn1 -- Diode3/RConn1 -- Diode2/LConn1
  C1/RConn1 -- Diode9/LConn1 -- Diode3/LConn1 -- R/RConn1 -- Vm2/LConn2
  Diode4/LConn1 -- Diode5/RConn1 -- A/RConn1
  IGBT/Diode1/LConn1 -- Diode10/RConn1 -- Diode6/LConn1 -- Diode7/RConn1
  Diode11/LConn1 -- IGBT/Diode1/RConn1 -- Diode8/LConn1 -- Diode9/RConn1
  Diode11/RConn1 -- B/RConn1 -- Diode10/LConn1

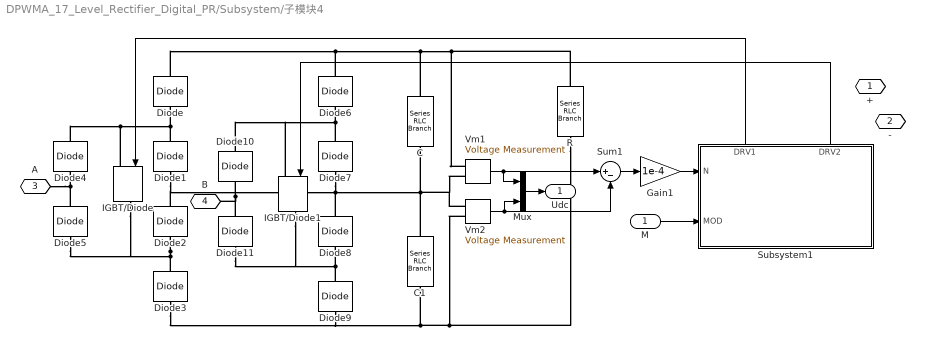
== system DPWMA_17_Level_Rectifier_Digital_PR/Subsystem/子模块4 ==
  M : Inport
  C : spsSeriesRLCBranchLib/Series RLC Branch  LConnTagsString=__new0  RConnTagsString=__new0  BranchType=C  Resistance=0  Inductance=0  SetiL0=off  InitialCurrent=0  Capacitance=4e-3  Setx0=on  InitialVoltage=850  Measurements=None
  C1 : spsSeriesRLCBranchLib/Series RLC Branch  LConnTagsString=__new0  RConnTagsString=__new0  BranchType=C  Resistance=0  Inductance=0  SetiL0=off  InitialCurrent=0  Capacitance=4e-3  Setx0=on  InitialVoltage=850  Measurements=None
  Diode{,1..3,6..9} (8 alike) : spsDiodeLib/Diode  Ron=0.001  Lon=0  Vf=1.8  IC=0  UseSnubber=0  Rs=5e6  Cs=2e-9  Measurements=off
  Diode{4..5,10..11} (4 alike) : spsDiodeLib/Diode  Ron=0.001  Lon=0  Vf=1  IC=0  UseSnubber=0  Rs=0.05  Cs=1e-8  Measurements=off
  Gain1 : Gain  Gain=1e-4
  IGBT/Diode : spsIGBTDiodeLib/IGBT//Diode  Ron=1e-3  Rs=1e5  Cs=inf  Measurements=off
  IGBT/Diode1 : spsIGBTDiodeLib/IGBT//Diode  Ron=1e-3  Rs=1e5  Cs=inf  Measurements=off
  Mux : Mux  Inputs=2
  R : spsSeriesRLCBranchLib/Series RLC Branch  LConnTagsString=__new0  RConnTagsString=__new0  BranchType=R  Resistance=30  Inductance=0  SetiL0=off  InitialCurrent=0  Capacitance=2e-3  Setx0=on  InitialVoltage=311  Measurements=None
  Subsystem1 : Subsystem
      settings: PortSchema="{\"entries\":[{\"content\":{\"sides\":[{\"content\":{\"connectorIds\":[\"In1\",\"In2\"]},\"type\":\"ConnectorPlacement.EquallySpacedRectSide\",\"uuid\":\"86aef1ad-fbca-44c0-97c4-c9d179baa788\"},{\"content\":{\"side\":\"RIGHT\"},\"type\":\"ConnectorPlacement.EquallySpacedRectSide\",\"uuid\":\"7b15a0f8-39b1-4cc5-afe7-a687626936eb\"},{\"content\":{\"connectorIds\":[\"Out1\",\"Out2\"],\"side\":\"TOP\"},\"type\":\"ConnectorPlacement.EquallySpacedRectSide\",\"uuid\":\"a58ec6d0-3129-4061-af12-e971b5e0e948\"}]},\"type\":\"ConnectorPlacement.EquallySpacedConnector\",\"uuid\":\"d3f7daee-0424-497d-bc41-11931290c6fe\"}],\"packageUris\":[\"http://schema.mathworks.com/mf0/Connector/R2020b\"],\"version\":\"1.0\"}"
  Sum1 : Sum  Inputs=|+-
  Vm1 : spsVoltageMeasurementLib/Voltage Measurement  PhasorSimulation=off  OutputType=Complex  PSBequivalent=0
  Vm2 : spsVoltageMeasurementLib/Voltage Measurement  PhasorSimulation=off  OutputType=Complex  PSBequivalent=0
  + : PMIOPort  Side=Left
  - : PMIOPort  Port=2  Side=Left
  A : PMIOPort  Port=3  Side=Right
  B : PMIOPort  Port=4  Side=Right
  Udc : Outport
  wires:
  Subsystem1/2(DRV2) -> IGBT/Diode1/1
  Subsystem1/1(DRV1) -> IGBT/Diode/1
  M/1 -> Subsystem1/2(MOD)
  Mux/1 -> Udc/1
  Gain1/1 -> Subsystem1/1(N)
  Sum1/1 -> Gain1/1
  Vm2/1 -> Sum1/2, Mux/2
  Vm1/1 -> Sum1/1, Mux/1
  connections:
  Diode10/LConn1 -- B/RConn1 -- Diode11/RConn1
  Diode9/RConn1 -- Diode8/LConn1 -- IGBT/Diode1/RConn1 -- Diode11/LConn1
  Diode7/RConn1 -- Diode6/LConn1 -- Diode10/RConn1 -- IGBT/Diode1/LConn1
  A/RConn1 -- Diode5/RConn1 -- Diode4/LConn1
  Vm2/LConn2 -- R/RConn1 -- Diode3/LConn1 -- Diode9/LConn1 -- C1/RConn1
  Diode2/LConn1 -- Diode3/RConn1 -- Diode5/LConn1 -- IGBT/Diode/RConn1
  Diode4/RConn1 -- IGBT/Diode/LConn1 -- Diode1/RConn1 -- Diode/LConn1
  Diode7/LConn1 -- Diode2/RConn1 -- Diode1/LConn1 -- C/RConn1 -- C1/LConn1 -- Vm2/LConn1 -- Vm1/LConn2 -- Diode8/RConn1
  Diode6/RConn1 -- Diode/RConn1 -- C/LConn1 -- R/LConn1 -- Vm1/LConn1
